simulink model "SNS_AirStep"  (R2025a)
settings: Solver=ode45  StartTime=0.0  StopTime=40  MaxStep=5e-4  RelTol=1e-3
PreLoadFcn:
  | I_h = 0.25;
  | b_h = 0.8;
  | I_k = 0.06;
  | b_k = 0.4;
  | m_t = 5;
  | l_c = 0.2;
  | m_s = 2;
  | l_cs = 0.22;
  | g = 9.81;
  | L0 = 0.185;
  | r_h = 0.045;
  | r_k = 0.035;
  | tauAct = 150;
  | Pmax = 620;
  | Fmax = 1148.3;
  | Rest = 0.2;
  | Kmax = 0.165;
libraries: SNS_Library x32
settings Model: Creator=Ben Bolen  LastModifiedBy=Ben Bolen

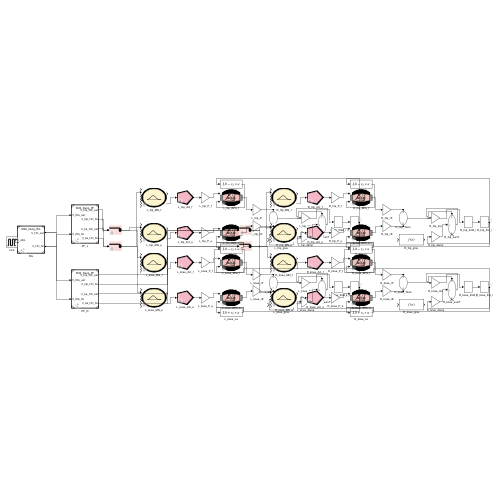
[thumbnail: Simulink's stored preview of the top-level diagram]
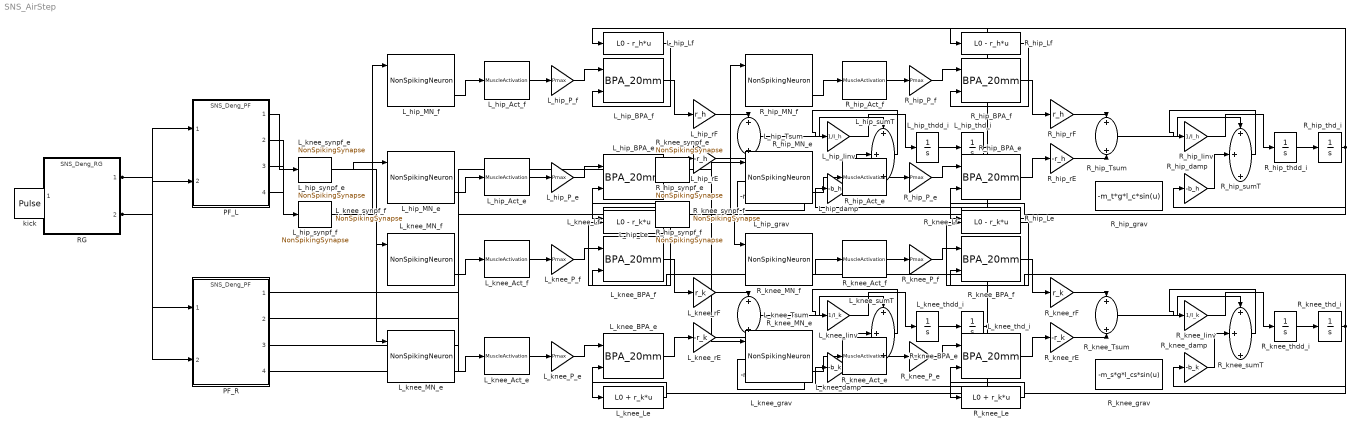
== system SNS_AirStep ==
  L_hip_Act_e : SNS_Library/MuscleActivation  tauAct=tauAct  A0=0
  L_hip_Act_f : SNS_Library/MuscleActivation  tauAct=tauAct  A0=0
  L_hip_BPA_e : SNS_Library/BPA_20mm  Rest=Rest  Kmax=Kmax  TendonL=0  FittingL=0
  L_hip_BPA_f : SNS_Library/BPA_20mm  Rest=Rest  Kmax=Kmax  TendonL=0  FittingL=0
  L_hip_Iinv : Gain  Gain=1/I_h
  L_hip_Le : Fcn  Expr=L0 + r_h*u
  L_hip_Lf : Fcn  Expr=L0 - r_h*u
  L_hip_MN_e : SNS_Library/NonSpikingNeuron  Vrest=-100  Gm=1  Cm=5  Thr=-60  Slope=10
  L_hip_MN_f : SNS_Library/NonSpikingNeuron  Vrest=-100  Gm=1  Cm=5  Thr=-60  Slope=10
  L_hip_P_e : Gain  Gain=Pmax
  L_hip_P_f : Gain  Gain=Pmax
  L_hip_Tsum : Sum
  L_hip_damp : Gain  Gain=-b_h
  L_hip_grav : Fcn  Expr=-m_t*g*l_c*sin(u)
  L_hip_rE : Gain  Gain=-r_h
  L_hip_rF : Gain  Gain=r_h
  L_hip_sumT : Sum  Inputs=+++
  L_hip_synpf_e : SNS_Library/NonSpikingSynapse  gmax=2.6563  Esyn=-10  ThrPre=-60  SlopePre=10
  L_hip_synpf_f : SNS_Library/NonSpikingSynapse  gmax=3.6325  Esyn=-10  ThrPre=-60  SlopePre=10
  L_hip_thd_i : Integrator
  L_hip_thdd_i : Integrator
  L_knee_Act_e : SNS_Library/MuscleActivation  tauAct=tauAct  A0=0
  L_knee_Act_f : SNS_Library/MuscleActivation  tauAct=tauAct  A0=0
  L_knee_BPA_e : SNS_Library/BPA_20mm  Rest=Rest  Kmax=Kmax  TendonL=0  FittingL=0
  L_knee_BPA_f : SNS_Library/BPA_20mm  Rest=Rest  Kmax=Kmax  TendonL=0  FittingL=0
  L_knee_Iinv : Gain  Gain=1/I_k
  L_knee_Le : Fcn  Expr=L0 + r_k*u
  L_knee_Lf : Fcn  Expr=L0 - r_k*u
  L_knee_MN_e : SNS_Library/NonSpikingNeuron  Vrest=-100  Gm=1  Cm=5  Thr=-60  Slope=10
  L_knee_MN_f : SNS_Library/NonSpikingNeuron  Vrest=-100  Gm=1  Cm=5  Thr=-60  Slope=10
  L_knee_P_e : Gain  Gain=Pmax
  L_knee_P_f : Gain  Gain=Pmax
  L_knee_Tsum : Sum
  L_knee_damp : Gain  Gain=-b_k
  L_knee_grav : Fcn  Expr=-m_s*g*l_cs*sin(u)
  L_knee_rE : Gain  Gain=-r_k
  L_knee_rF : Gain  Gain=r_k
  L_knee_sumT : Sum  Inputs=+++
  L_knee_synpf_e : SNS_Library/NonSpikingSynapse  gmax=4.9296  Esyn=-10  ThrPre=-60  SlopePre=10
  L_knee_synpf_f : SNS_Library/NonSpikingSynapse  gmax=1.5165  Esyn=-10  ThrPre=-60  SlopePre=10
  L_knee_thd_i : Integrator
  L_knee_thdd_i : Integrator
  PF_L : ModelReference  ModelNameDialog=SNS_Deng_PF.slx  SimulationMode=Normal  ModelReferenceVersion=1.1
  PF_R : ModelReference  ModelNameDialog=SNS_Deng_PF.slx  SimulationMode=Normal  ModelReferenceVersion=1.1
  RG : ModelReference  ModelNameDialog=SNS_Deng_RG.slx  SimulationMode=Normal  ModelReferenceVersion=1.1
  R_hip_Act_e : SNS_Library/MuscleActivation  tauAct=tauAct  A0=0
  R_hip_Act_f : SNS_Library/MuscleActivation  tauAct=tauAct  A0=0
  R_hip_BPA_e : SNS_Library/BPA_20mm  Rest=Rest  Kmax=Kmax  TendonL=0  FittingL=0
  R_hip_BPA_f : SNS_Library/BPA_20mm  Rest=Rest  Kmax=Kmax  TendonL=0  FittingL=0
  R_hip_Iinv : Gain  Gain=1/I_h
  R_hip_Le : Fcn  Expr=L0 + r_h*u
  R_hip_Lf : Fcn  Expr=L0 - r_h*u
  R_hip_MN_e : SNS_Library/NonSpikingNeuron  Vrest=-100  Gm=1  Cm=5  Thr=-60  Slope=10
  R_hip_MN_f : SNS_Library/NonSpikingNeuron  Vrest=-100  Gm=1  Cm=5  Thr=-60  Slope=10
  R_hip_P_e : Gain  Gain=Pmax
  R_hip_P_f : Gain  Gain=Pmax
  R_hip_Tsum : Sum
  R_hip_damp : Gain  Gain=-b_h
  R_hip_grav : Fcn  Expr=-m_t*g*l_c*sin(u)
  R_hip_rE : Gain  Gain=-r_h
  R_hip_rF : Gain  Gain=r_h
  R_hip_sumT : Sum  Inputs=+++
  R_hip_synpf_e : SNS_Library/NonSpikingSynapse  gmax=2.6563  Esyn=-10  ThrPre=-60  SlopePre=10
  R_hip_synpf_f : SNS_Library/NonSpikingSynapse  gmax=3.6325  Esyn=-10  ThrPre=-60  SlopePre=10
  R_hip_thd_i : Integrator
  R_hip_thdd_i : Integrator
  R_knee_Act_e : SNS_Library/MuscleActivation  tauAct=tauAct  A0=0
  R_knee_Act_f : SNS_Library/MuscleActivation  tauAct=tauAct  A0=0
  R_knee_BPA_e : SNS_Library/BPA_20mm  Rest=Rest  Kmax=Kmax  TendonL=0  FittingL=0
  R_knee_BPA_f : SNS_Library/BPA_20mm  Rest=Rest  Kmax=Kmax  TendonL=0  FittingL=0
  R_knee_Iinv : Gain  Gain=1/I_k
  R_knee_Le : Fcn  Expr=L0 + r_k*u
  R_knee_Lf : Fcn  Expr=L0 - r_k*u
  R_knee_MN_e : SNS_Library/NonSpikingNeuron  Vrest=-100  Gm=1  Cm=5  Thr=-60  Slope=10
  R_knee_MN_f : SNS_Library/NonSpikingNeuron  Vrest=-100  Gm=1  Cm=5  Thr=-60  Slope=10
  R_knee_P_e : Gain  Gain=Pmax
  R_knee_P_f : Gain  Gain=Pmax
  R_knee_Tsum : Sum
  R_knee_damp : Gain  Gain=-b_k
  R_knee_grav : Fcn  Expr=-m_s*g*l_cs*sin(u)
  R_knee_rE : Gain  Gain=-r_k
  R_knee_rF : Gain  Gain=r_k
  R_knee_sumT : Sum  Inputs=+++
  R_knee_synpf_e : SNS_Library/NonSpikingSynapse  gmax=4.9296  Esyn=-10  ThrPre=-60  SlopePre=10
  R_knee_synpf_f : SNS_Library/NonSpikingSynapse  gmax=1.5165  Esyn=-10  ThrPre=-60  SlopePre=10
  R_knee_thd_i : Integrator
  R_knee_thdd_i : Integrator
  kick : DiscretePulseGenerator  PulseType=Time based  Amplitude=10  Period=500  PulseWidth=0.002  PhaseDelay=0.1
  wires:
  kick/1 -> RG/1
  RG/1 -> PF_L/1, PF_R/2
  RG/2 -> PF_L/2, PF_R/1
  L_hip_MN_f/2 -> L_hip_Act_f/1
  L_hip_MN_e/2 -> L_hip_Act_e/1
  L_hip_Act_f/1 -> L_hip_P_f/1
  L_hip_Act_e/1 -> L_hip_P_e/1
  L_hip_P_f/1 -> L_hip_BPA_f/1
  L_hip_P_e/1 -> L_hip_BPA_e/1
  L_hip_BPA_f/1 -> L_hip_rF/1
  L_hip_BPA_e/1 -> L_hip_rE/1
  L_hip_rF/1 -> L_hip_Tsum/1
  L_hip_rE/1 -> L_hip_Tsum/2
  L_hip_Tsum/1 -> L_hip_sumT/1
  L_hip_thd_i/1 -> L_hip_damp/1, L_hip_Lf/1, L_hip_Le/1
  L_hip_damp/1 -> L_hip_sumT/2
  L_hip_sumT/1 -> L_hip_Iinv/1
  L_hip_Iinv/1 -> L_hip_thdd_i/1
  L_hip_thdd_i/1 -> L_hip_thd_i/1
  L_hip_Lf/1 -> L_hip_BPA_f/2
  L_hip_Le/1 -> L_hip_BPA_e/2
  L_knee_MN_f/2 -> L_knee_Act_f/1
  L_knee_MN_e/2 -> L_knee_Act_e/1
  L_knee_Act_f/1 -> L_knee_P_f/1
  L_knee_Act_e/1 -> L_knee_P_e/1
  L_knee_P_f/1 -> L_knee_BPA_f/1
  L_knee_P_e/1 -> L_knee_BPA_e/1
  L_knee_BPA_f/1 -> L_knee_rF/1
  L_knee_BPA_e/1 -> L_knee_rE/1
  L_knee_rF/1 -> L_knee_Tsum/1
  L_knee_rE/1 -> L_knee_Tsum/2
  L_knee_Tsum/1 -> L_knee_sumT/1
  L_knee_thd_i/1 -> L_knee_damp/1, L_knee_Lf/1, L_knee_Le/1
  L_knee_damp/1 -> L_knee_sumT/2
  L_knee_sumT/1 -> L_knee_Iinv/1
  L_knee_Iinv/1 -> L_knee_thdd_i/1
  L_knee_thdd_i/1 -> L_knee_thd_i/1
  L_knee_Lf/1 -> L_knee_BPA_f/2
  L_knee_Le/1 -> L_knee_BPA_e/2
  R_hip_MN_f/2 -> R_hip_Act_f/1
  R_hip_MN_e/2 -> R_hip_Act_e/1
  R_hip_Act_f/1 -> R_hip_P_f/1
  R_hip_Act_e/1 -> R_hip_P_e/1
  R_hip_P_f/1 -> R_hip_BPA_f/1
  R_hip_P_e/1 -> R_hip_BPA_e/1
  R_hip_BPA_f/1 -> R_hip_rF/1
  R_hip_BPA_e/1 -> R_hip_rE/1
  R_hip_rF/1 -> R_hip_Tsum/1
  R_hip_rE/1 -> R_hip_Tsum/2
  R_hip_Tsum/1 -> R_hip_sumT/1
  R_hip_thd_i/1 -> R_hip_damp/1, R_hip_Lf/1, R_hip_Le/1
  R_hip_damp/1 -> R_hip_sumT/2
  R_hip_sumT/1 -> R_hip_Iinv/1
  R_hip_Iinv/1 -> R_hip_thdd_i/1
  R_hip_thdd_i/1 -> R_hip_thd_i/1
  R_hip_Lf/1 -> R_hip_BPA_f/2
  R_hip_Le/1 -> R_hip_BPA_e/2
  R_knee_MN_f/2 -> R_knee_Act_f/1
  R_knee_MN_e/2 -> R_knee_Act_e/1
  R_knee_Act_f/1 -> R_knee_P_f/1
  R_knee_Act_e/1 -> R_knee_P_e/1
  R_knee_P_f/1 -> R_knee_BPA_f/1
  R_knee_P_e/1 -> R_knee_BPA_e/1
  R_knee_BPA_f/1 -> R_knee_rF/1
  R_knee_BPA_e/1 -> R_knee_rE/1
  R_knee_rF/1 -> R_knee_Tsum/1
  R_knee_rE/1 -> R_knee_Tsum/2
  R_knee_Tsum/1 -> R_knee_sumT/1
  R_knee_thd_i/1 -> R_knee_damp/1, R_knee_Lf/1, R_knee_Le/1
  R_knee_damp/1 -> R_knee_sumT/2
  R_knee_sumT/1 -> R_knee_Iinv/1
  R_knee_Iinv/1 -> R_knee_thdd_i/1
  R_knee_thdd_i/1 -> R_knee_thd_i/1
  R_knee_Lf/1 -> R_knee_BPA_f/2
  R_knee_Le/1 -> R_knee_BPA_e/2
  PF_L/1 -> L_hip_synpf_e/1
  L_hip_synpf_e/1 -> L_hip_MN_e/2
  PF_L/2 -> L_hip_synpf_f/1
  L_hip_synpf_f/1 -> L_hip_MN_f/2
  PF_L/3 -> L_knee_synpf_e/1
  L_knee_synpf_e/1 -> L_knee_MN_e/2
  PF_L/4 -> L_knee_synpf_f/1
  L_knee_synpf_f/1 -> L_knee_MN_f/2
  PF_R/1 -> R_hip_synpf_e/1
  R_hip_synpf_e/1 -> R_hip_MN_e/2
  PF_R/2 -> R_hip_synpf_f/1
  R_hip_synpf_f/1 -> R_hip_MN_f/2
  PF_R/3 -> R_knee_synpf_e/1
  R_knee_synpf_e/1 -> R_knee_MN_e/2
  PF_R/4 -> R_knee_synpf_f/1
  R_knee_synpf_f/1 -> R_knee_MN_f/2
